simulink model "SMC_bicycle_sim"  (R2026b)
settings: Solver=VariableStepAuto  StopTime=10  MaxStep=0.01
values from neighbouring files (symbols this model uses):
  A = zeros(2,2)    [SMC_bicycle.m]
  A_ = [0,-C ... (first row only)    [SMC_bicycle.m]
  B = zeros(2,1)    [SMC_bicycle.m]
  C = [1,0]    [SMC_bicycle.m]
  E = zeros(2,1)    [SMC_bicycle.m]
  G_ = [eye(1);0;0]    [SMC_bicycle.m]
  invSB_ = inv(S*B_)    [SMC_bicycle.m]
  k1 = 12    [SMC_bicycle.m]
  k2 = 0.05    [SMC_bicycle.m]
  S = [F_,eye(1)]    [SMC_bicycle.m]
  ToRad = pi/180    (= 0.0174532925199)    [SMC_bicycle.m]
settings Model: Creator=TominoShun  LastModifiedBy=富野

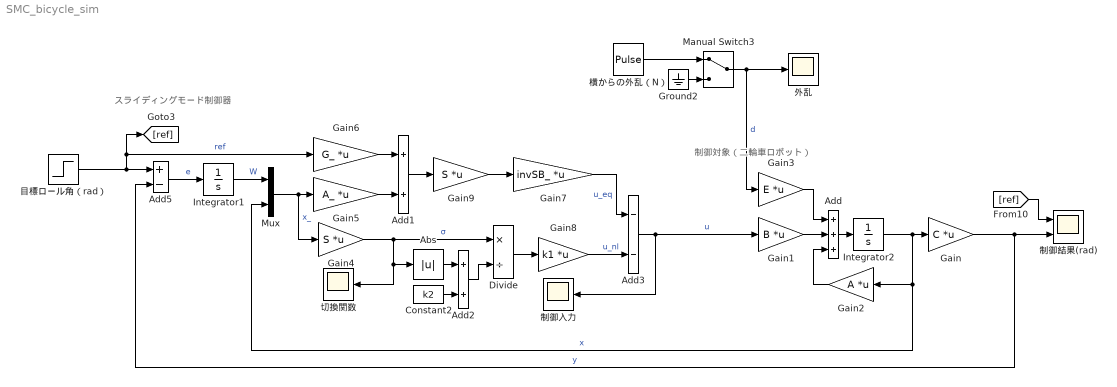
== system SMC_bicycle_sim ==
  note: 制御対象（二輪車ロボット）
  note: スライディングモード制御器
  Abs : Abs  SaturateOnIntegerOverflow=off
  Add : Sum  Inputs=+++
  Add1 : Sum
  Add2 : Sum
  Add3 : Sum  Inputs=--
  Add5 : Sum  Inputs=+-
  Constant2 : Constant  Value=k2
  Divide : Product  Inputs=*/
  Gain : Gain  Gain=C  Multiplication=Matrix(K*u)
  Gain1 : Gain  Gain=B  Multiplication=Matrix(K*u)
  Gain2 : Gain  Gain=A  Multiplication=Matrix(K*u)
  Gain3 : Gain  Gain=E  Multiplication=Matrix(K*u)
  Gain4 : Gain  Gain=S  Multiplication=Matrix(K*u)
  Gain5 : Gain  Gain=A_  Multiplication=Matrix(K*u)
  Gain6 : Gain  Gain=G_  Multiplication=Matrix(K*u)
  Gain7 : Gain  Gain=invSB_  Multiplication=Matrix(K*u)
  Gain8 : Gain  Gain=k1  Multiplication=Matrix(K*u)
  Gain9 : Gain  Gain=S  Multiplication=Matrix(K*u)
  Ground2 : Ground
  Integrator1 : Integrator
  Integrator2 : Integrator
  Manual Switch3 : ManualSwitch
  Mux : Mux  Inputs=2
  切換関数 : Scope
      settings: ActiveDisplayYMinimum=-0.0016003763875934564  ActiveDisplayYMaximum=0.0001778195986242934
  制御入力 : Scope
      settings: TimeUnits=Metric (based on Time Span)  ActiveDisplayYMinimum=-0.64859130253224206  ActiveDisplayYMaximum=0.30730812294303644  YLabel=外乱(N)  DataLoggingVariableName=ScopeData3
  制御結果(rad) : Scope  NumInputPorts=2
      settings: TimeUnits=Metric (based on Time Span)  ActiveDisplayYMinimum=-0.36294487149381238  ActiveDisplayYMaximum=0.31403987555345086  YLabel=ロール角(rad)  DataLoggingVariableName=ScopeData2
  外乱 : Scope
      settings: TimeUnits=Metric (based on Time Span)  ActiveDisplayYMinimum=-0.12499999999999997  ActiveDisplayYMaximum=1.125  YLabel=外乱(N)
  横からの外乱（N） : DiscretePulseGenerator  PulseType=Time based  Period=10  PulseWidth=10  PhaseDelay=5
  目標ロール角（rad） : Step  Time=2  FinalValue=10*ToRad  SampleTime=0
  wires:
  Integrator1/1 -> Mux/1  "W"
  Add5/1 -> Integrator1/1  "e"
  目標ロール角（rad）/1 -> Gain6/1, [ref], Add5/1  "ref"
  Ground2/1 -> Manual Switch3/2
  Manual Switch3/1 -> 外乱/1, Gain3/1  "d"
  横からの外乱（N）/1 -> Manual Switch3/1
  Gain2/1 -> Add/3
  Add3/1 -> Gain1/1, 制御入力/1  "u"
  Add/1 -> Integrator2/1
  Integrator2/1 -> Gain2/1, Mux/2, Gain/1  "x"
  Gain1/1 -> Add/2
  Gain/1 -> 制御結果(rad)/2, Add5/2  "y"
  Gain3/1 -> Add/1
  Mux/1 -> Gain4/1, Gain5/1  "x_"
  Gain4/1 -> 切換関数/1, Abs/1, Divide/1  "σ"
  Gain6/1 -> Add1/1
  Gain5/1 -> Add1/2
  Add1/1 -> Gain9/1
  Constant2/1 -> Add2/2
  Abs/1 -> Add2/1
  Add2/1 -> Divide/2
  Divide/1 -> Gain8/1
  Gain8/1 -> Add3/2  "u_nl"
  Gain7/1 -> Add3/1  "u_eq"
  [ref] -> 制御結果(rad)/1
  Gain9/1 -> Gain7/1
